simulink model "TLLTD_V1"  (R2025b)
settings: Solver=VariableStepAuto  StartTime=0.0  StopTime=10.0  RelTol=1e-3
model workspace (MAT data in the model file):
  Var = 0
  g = 9.81
values from neighbouring files (symbols this model uses):
  Track_Width = 1.00    (= 1)    [LoadTransferSimulationRevised.m]
undefined symbols (not defined in the file or in its folder): Front_Wheelbase, Rear_Wheelbase
settings Model: Creator=jakub  LastModifiedBy=jakub

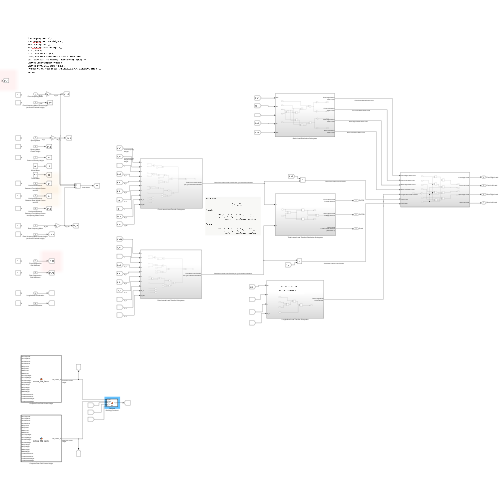
[thumbnail: Simulink's stored preview of the top-level diagram]
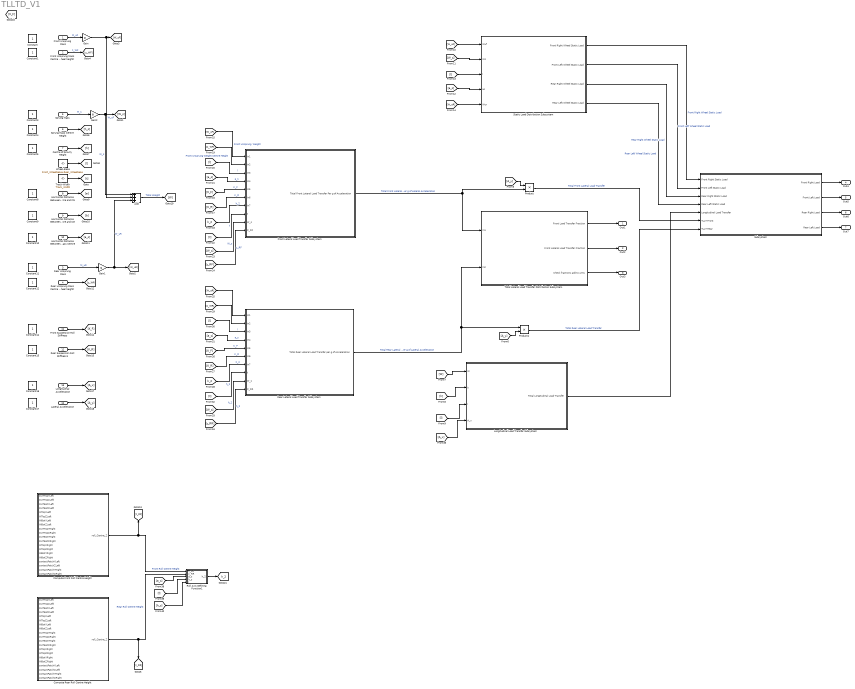
== system TLLTD_V1 ==
  Front Unsprung Mass : Inport
  Front Unsprung Mass Centre height (at centre of wheel height) : Inport  Port=2
  Rear Unsprung Mass : Inport  Port=3
  Rear Unsprung Mass Centre height (at centre of wheel height) : Inport  Port=4
  Sprung Mass : Inport  Port=5
  Sprung Mass Centre Height : Inport  Port=6
  Centre of Gravity Height : Inport  Port=7
  Horizontal Distance Between Front Wheel Centre and CG : Inport  Port=8
  Horizontal Distance Between Rear Wheel Centre and CG : Inport  Port=9
  Horizontal Distance Between Front Wheel Centre and Sprung Mass Centre : Inport  Port=10
  Front Suspension Roll Stiffness : Inport  Port=11
  Rear Suspension Roll Stiffness1 : Inport  Port=12
  Longitudinal Acceleration : Inport  Port=13
  Lateral Acceleration : Inport  Port=14
  Add : Sum  Inputs=+++
  Compute Front Roll Centre Height : MATLAB Function  TreatAsAtomicUnit=on
  Compute Rear Roll Centre Height : MATLAB Function  TreatAsAtomicUnit=on
  Constant{,1,3..5,8..12,14..17} (14 alike) : Constant
  Front Lateral Load Transfer Subsystem : Subsystem
  Gain : Gain  Gain=g
  Gain1 : Gain  Gain=g
  Gain2 : Gain  Gain=g
  Longitudinal Load Transfer Subsystem : Subsystem
  Product : Product
  Product1 : Product
  Rear Lateral Load Transfer Subsystem : Subsystem
  Roll Axis Defining Function1 : MATLAB Function  TreatAsAtomicUnit=on
  Static Load Distribution Subsystem : Subsystem
  Subsystem : Subsystem
  Total Lateral Load Transfer Distribution Subsystem : Subsystem
  Track-Width : Constant  Value=Track_Width
  Wheel-Base : Constant  Value=Front_Wheelbase+Rear_Wheelbase
  Out1 : Outport  SignalName=TLLTDF
  Out2 : Outport  Port=2  SignalName=TLLTDR
  Out3 : Outport  Port=3  SignalName=Check
  Out4 : Outport  Port=4  SignalName=Front Right Load
  Out5 : Outport  Port=5  SignalName=Front Left Load
  Out6 : Outport  Port=6  SignalName=Rear Right Load
  Out7 : Outport  Port=7  SignalName=Rear Left Load
  tag scope: h_2=global
  wires:
  Gain/1 -> Add/2, [W_uF]  "W_uF"
  Rear Unsprung Mass/1 -> Gain1/1  "M_uR"
  Gain1/1 -> Add/3, [W_uR]  "W_uR"
  Sprung Mass/1 -> Gain2/1  "M_s"
  Gain2/1 -> Add/1, [W_s]  "W_s"
  Track-Width/1 -> [t]
  Front Unsprung Mass/1 -> Gain/1  "M_uF"
  Front Unsprung Mass Centre height (at centre of wheel height)/1 -> [z_WF]  "z_WF"
  Sprung Mass Centre Height/1 -> [h_s]
  Centre of Gravity Height/1 -> [h]
  Wheel-Base/1 -> [l]
  Horizontal Distance Between Front Wheel Centre and CG/1 -> [a]
  Horizontal Distance Between Rear Wheel Centre and CG/1 -> [b]
  Horizontal Distance Between Front Wheel Centre and Sprung Mass Centre/1 -> [a_s]
  Rear Unsprung Mass Centre height (at centre of wheel height)/1 -> [z_WR]
  Front Suspension Roll Stiffness/1 -> [K_F]
  Rear Suspension Roll Stiffness1/1 -> [K_R]
  Total Lateral Load Transfer Distribution Subsystem/1(Front Load Transfer Fraction) -> Out1/1
  Total Lateral Load Transfer Distribution Subsystem/2(Front Lateral Load Transfer Fraction) -> Out2/1
  Front Lateral Load Transfer Subsystem/1(Total Front Lateral Load Transfer Per g of Acceleration) -> Total Lateral Load Transfer Distribution Subsystem/1(In1), Product/2  "Total Front Lateral Load Transfer Per g of Lateral Acceleration"
  Rear Lateral Load Transfer Subsystem/1(Total Rear Lateral Load Transfer per g of Acceleration) -> Total Lateral Load Transfer Distribution Subsystem/2(In2), Product1/1  "Total Rear Lateral Load Transfer per g of Lateral Acceleration"
  Total Lateral Load Transfer Distribution Subsystem/3(Check fractions add to unity) -> Out3/1
  Static Load Distribution Subsystem/1(Front Right Wheel Static Load) -> Subsystem/1(Front Right Static Load)  "Front Right Wheel Static Load"
  Static Load Distribution Subsystem/2(Front Left Wheel Static Load) -> Subsystem/2(Front Left Static Load)  "Front Left Wheel Static Load"
  Static Load Distribution Subsystem/3(Rear Right Wheel Static Load) -> Subsystem/3(Rear Right Static Load)  "Rear Right Wheel Static Load"
  Static Load Distribution Subsystem/4(Rear Left Wheel Static Load) -> Subsystem/4(Rear Left Static Load)  "Rear Left Wheel Static Load"
  Longitudinal Acceleration/1 -> [A_x]
  Lateral Acceleration/1 -> [A_y]
  Add/1 -> [W]  "Total Weight"
  [A_y] -> Product/1
  Product/1 -> Subsystem/6(TLLT Front)  "Total Front Lateral Load Transfer"
  [A_y] -> Product1/2
  Product1/1 -> Subsystem/7(TLLT Rear)  "Total Rear Lateral Load Transfer"
  Longitudinal Load Transfer Subsystem/1(Total Longitudinal Load Transfer) -> Subsystem/5(Longitudinal Load Transfer)
  Subsystem/1(Front Right Load) -> Out4/1
  Subsystem/2(Front Left Load) -> Out5/1
  Subsystem/3(Rear Right Load) -> Out6/1
  Subsystem/4(Rear Left Load) -> Out7/1
  [W] -> Longitudinal Load Transfer Subsystem/1(W)
  [h] -> Longitudinal Load Transfer Subsystem/2(h)
  [l] -> Longitudinal Load Transfer Subsystem/3(l)
  [W_uF] -> Static Load Distribution Subsystem/1(Wuf)
  [W_s] -> Static Load Distribution Subsystem/2(Ws)
  [l] -> Static Load Distribution Subsystem/3(l)
  [a_s] -> Static Load Distribution Subsystem/4(as)
  [W_uR] -> Static Load Distribution Subsystem/5(Wur)
  [t] -> Front Lateral Load Transfer Subsystem/8(t)  "t"
  [W_s] -> Front Lateral Load Transfer Subsystem/9(W_s)  "W_s"
  [z_RF] -> Front Lateral Load Transfer Subsystem/10(Z_RF)  "z_RF"
  [h_2] -> Front Lateral Load Transfer Subsystem/7(In7)  "h_2"
  [K_R] -> Front Lateral Load Transfer Subsystem/6(In6)  "K_R"
  [K_F] -> Front Lateral Load Transfer Subsystem/5(In5)  "K_F"
  [a_s] -> Front Lateral Load Transfer Subsystem/4(In4)  "a_s"
  [l] -> Front Lateral Load Transfer Subsystem/3(In3)  "l"
  [z_WF] -> Front Lateral Load Transfer Subsystem/2(In2)  "Front Unsprung Weight Centre Height"
  [W_uF] -> Front Lateral Load Transfer Subsystem/1(In1)  "Front Unsprung  Weight"
  [W_s] -> Rear Lateral Load Transfer Subsystem/9(W_s)  "h_2"
  [t] -> Rear Lateral Load Transfer Subsystem/8(t)  "h_2"
  [K_F] -> Rear Lateral Load Transfer Subsystem/5(In5)  "K_F"
  [h_2] -> Rear Lateral Load Transfer Subsystem/7(In7)  "h_2"
  [K_R] -> Rear Lateral Load Transfer Subsystem/6(In6)  "K_R"
  [W_uR] -> Rear Lateral Load Transfer Subsystem/1(In1)
  [a_s] -> Rear Lateral Load Transfer Subsystem/4(In4)  "a_s"
  [l] -> Rear Lateral Load Transfer Subsystem/3(In3)  "l"
  [z_RR] -> Rear Lateral Load Transfer Subsystem/10(Z_RR)  "h_2"
  [z_WR] -> Rear Lateral Load Transfer Subsystem/2(In2)
  [A_x] -> Longitudinal Load Transfer Subsystem/4(A_x)
  Compute Rear Roll Centre Height/1(roll_Centre_Z) -> [z_RR], Roll Axis Defining Function1/2(z_RR)  "Rear Roll Centre Height"
  Roll Axis Defining Function1/1(h_2) -> [h_2]
  [a_s] -> Roll Axis Defining Function1/3(a_s)
  [h_s] -> Roll Axis Defining Function1/5(l)
  [l] -> Roll Axis Defining Function1/4(h_s)
  Compute Front Roll Centre Height/1(roll_Centre_Z) -> [z_RF], Roll Axis Defining Function1/1(z_RF)  "Front Roll Centre Height"

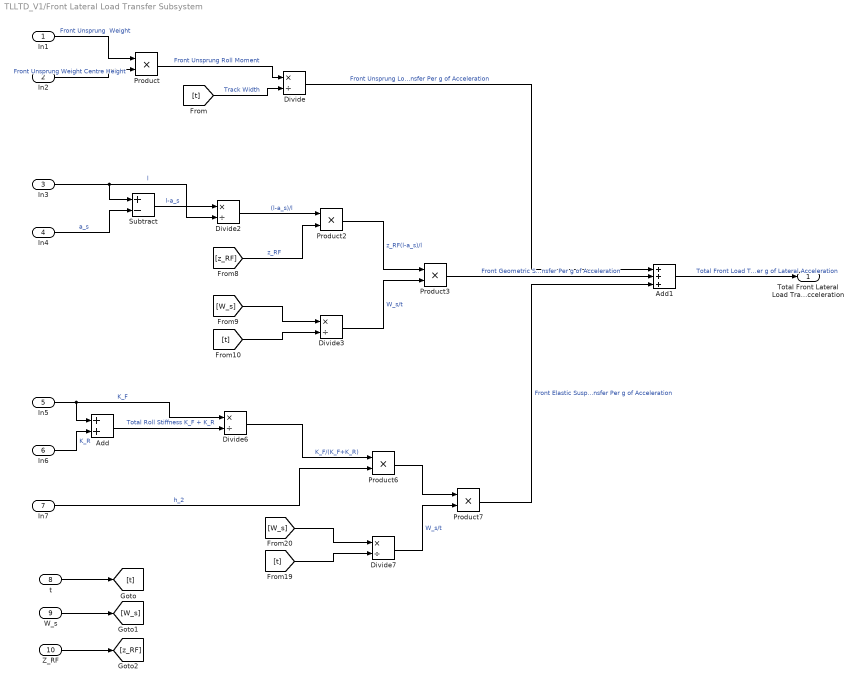
== system TLLTD_V1/Front Lateral Load Transfer Subsystem ==
  In1 : Inport
  In2 : Inport  Port=2
  In3 : Inport  Port=3
  In4 : Inport  Port=4
  In5 : Inport  Port=5
  In6 : Inport  Port=6
  In7 : Inport  Port=7
  t : Inport  Port=8
  W_s : Inport  Port=9
  Z_RF : Inport  Port=10
  Add : Sum
  Add1 : Sum  Inputs=+++
  Divide{,2..3,6..7} (5 alike) : Product  Inputs=*/
  Product{,2..3,6..7} (5 alike) : Product
  Subtract : Sum  Inputs=+-
  Total Front Lateral Load Transfer Per g of Acceleration : Outport
  wires:
  In1/1 -> Product/1  "Front Unsprung  Weight"
  Product7/1 -> Add1/3  "Front Elastic Suspended Load Transfer Per g of Acceleration"
  Divide3/1 -> Product3/2  "W_s/t"
  In2/1 -> Product/2  "Front Unsprung Weight Centre Height"
  [W_s] -> Divide3/1
  In7/1 -> Product6/2  "h_2"
  Product/1 -> Divide/1  "Front Unsprung Roll Moment"
  In3/1 -> Divide2/2, Subtract/1  "l"
  Divide/1 -> Add1/1  "Front Unsprung Load Transfer Per g of Acceleration"
  [W_s] -> Divide7/1
  In5/1 -> Divide6/1, Add/1  "K_F"
  [t] -> Divide3/2
  In4/1 -> Subtract/2  "a_s"
  [z_RF] -> Product2/2  "z_RF"
  Add/1 -> Divide6/2  "Total Roll Stiffness K_F + K_R"
  Divide2/1 -> Product2/1  "(l-a_s)/l"
  Add1/1 -> Total Front Lateral Load Transfer Per g of Acceleration/1  "Total Front Load Transfer per g of Lateral Acceleration"
  Product2/1 -> Product3/1  "z_RF(l-a_s)/l"
  Subtract/1 -> Divide2/1  "l-a_s"
  Product6/1 -> Product7/1
  [t] -> Divide7/2
  [t] -> Divide/2  "Track Width"
  Divide7/1 -> Product7/2  "W_s/t"
  Divide6/1 -> Product6/1  "K_F/(K_F+K_R)"
  In6/1 -> Add/2  "K_R"
  Product3/1 -> Add1/2  "Front Geometric Suspended Load Transfer Per g of Acceleration"
  t/1 -> [t]
  W_s/1 -> [W_s]
  Z_RF/1 -> [z_RF]

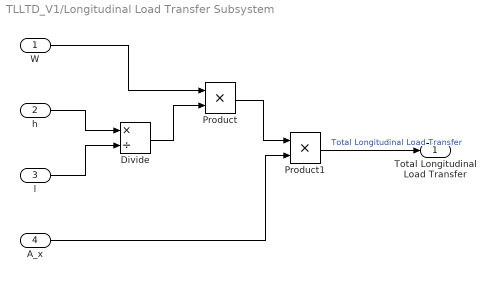
== system TLLTD_V1/Longitudinal Load Transfer Subsystem ==
  W : Inport
  h : Inport  Port=2
  l : Inport  Port=3
  A_x : Inport  Port=4
  Divide : Product  Inputs=*/
  Product : Product
  Product1 : Product
  Total Longitudinal Load Transfer : Outport
  wires:
  Product/1 -> Product1/1
  Product1/1 -> Total Longitudinal Load Transfer/1  "Total Longitudinal Load Transfer"
  Divide/1 -> Product/2
  A_x/1 -> Product1/2
  W/1 -> Product/1
  h/1 -> Divide/1
  l/1 -> Divide/2

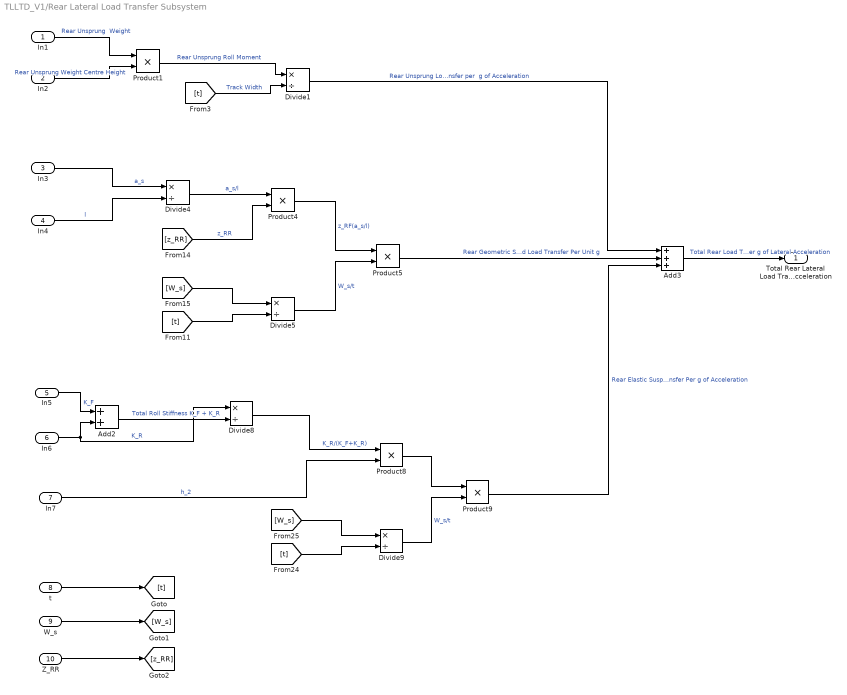
== system TLLTD_V1/Rear Lateral Load Transfer Subsystem ==
  In1 : Inport
  In2 : Inport  Port=2
  In3 : Inport  Port=3
  In4 : Inport  Port=4
  In5 : Inport  Port=5
  In6 : Inport  Port=6
  In7 : Inport  Port=7
  t : Inport  Port=8
  W_s : Inport  Port=9
  Z_RR : Inport  Port=10
  Add2 : Sum
  Add3 : Sum  Inputs=+++
  Divide{1,4..5,8..9} (5 alike) : Product  Inputs=*/
  Product{1,4..5,8..9} (5 alike) : Product
  Total Rear Lateral Load Transfer per g of Acceleration : Outport
  wires:
  Divide4/1 -> Product4/1  "a_s/l"
  Add2/1 -> Divide8/2  "Total Roll Stiffness K_F + K_R"
  [t] -> Divide9/2
  Divide8/1 -> Product8/1  "K_R/(K_F+K_R)"
  [W_s] -> Divide9/1
  Product8/1 -> Product9/1
  Add3/1 -> Total Rear Lateral Load Transfer per g of Acceleration/1  "Total Rear Load Transfer Per g of Lateral Acceleration"
  In5/1 -> Add2/1  "K_F"
  In6/1 -> Divide8/1, Add2/2  "K_R"
  Product9/1 -> Add3/3  "Rear Elastic Suspended Load Transfer Per g of Acceleration"
  In7/1 -> Product8/2  "h_2"
  Divide1/1 -> Add3/1  "Rear Unsprung Load Transfer per  g of Acceleration"
  In3/1 -> Divide4/1  "a_s"
  [t] -> Divide1/2  "Track Width"
  Product1/1 -> Divide1/1  "Rear Unsprung Roll Moment"
  In2/1 -> Product1/2  "Rear Unsprung Weight Centre Height"
  In1/1 -> Product1/1  "Rear Unsprung  Weight"
  Divide9/1 -> Product9/2  "W_s/t"
  [t] -> Divide5/2
  Product5/1 -> Add3/2  "Rear Geometric Suspended Load Transfer Per Unit g"
  [z_RR] -> Product4/2  "z_RR"
  Product4/1 -> Product5/1  "z_RF(a_s/l)"
  In4/1 -> Divide4/2  "l"
  Divide5/1 -> Product5/2  "W_s/t"
  [W_s] -> Divide5/1
  t/1 -> [t]
  W_s/1 -> [W_s]
  Z_RR/1 -> [z_RR]

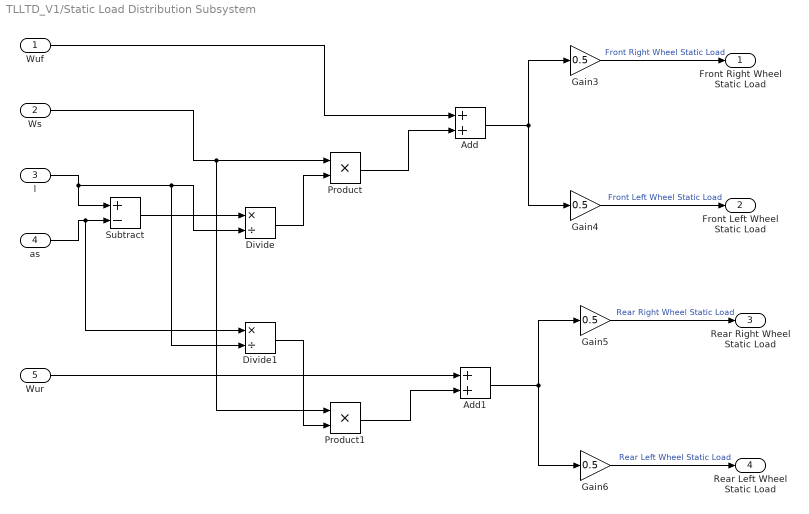
== system TLLTD_V1/Static Load Distribution Subsystem ==
  Wuf : Inport
  Ws : Inport  Port=2
  l : Inport  Port=3
  as : Inport  Port=4
  Wur : Inport  Port=5
  Add : Sum
  Add1 : Sum
  Divide : Product  Inputs=*/
  Divide1 : Product  Inputs=*/
  Gain{3..6} (4 alike) : Gain  Gain=0.5
  Product : Product
  Product1 : Product
  Subtract : Sum  Inputs=+-
  Front Right Wheel Static Load : Outport
  Front Left Wheel Static Load : Outport  Port=2
  Rear Right Wheel Static Load : Outport  Port=3
  Rear Left Wheel Static Load : Outport  Port=4
  wires:
  Gain6/1 -> Rear Left Wheel Static Load/1  "Rear Left Wheel Static Load"
  l/1 -> Divide1/2, Divide/2, Subtract/1
  Add1/1 -> Gain6/1, Gain5/1
  Product/1 -> Add/2
  Gain5/1 -> Rear Right Wheel Static Load/1  "Rear Right Wheel Static Load"
  Ws/1 -> Product1/1, Product/1
  as/1 -> Divide1/1, Subtract/2
  Add/1 -> Gain3/1, Gain4/1
  Product1/1 -> Add1/2
  Divide1/1 -> Product1/2
  Divide/1 -> Product/2
  Gain3/1 -> Front Right Wheel Static Load/1  "Front Right Wheel Static Load"
  Subtract/1 -> Divide/1
  Wuf/1 -> Add/1
  Gain4/1 -> Front Left Wheel Static Load/1  "Front Left Wheel Static Load"
  Wur/1 -> Add1/1

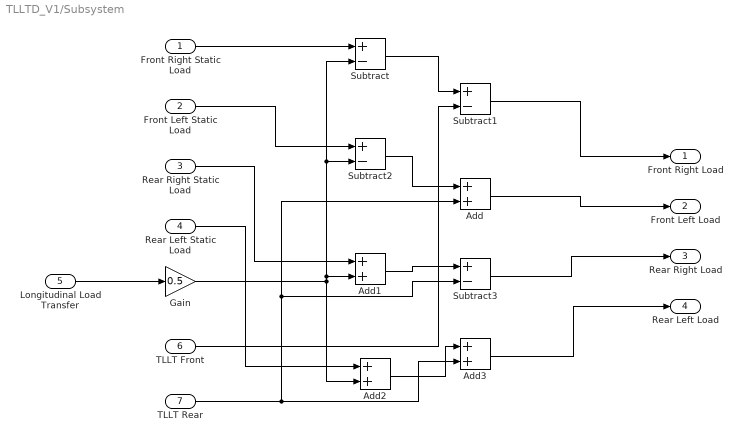
== system TLLTD_V1/Subsystem ==
  Front Right Static Load : Inport
  Front Left Static Load : Inport  Port=2
  Rear Right Static Load : Inport  Port=3
  Rear Left Static Load : Inport  Port=4
  Longitudinal Load Transfer : Inport  Port=5
  TLLT Front : Inport  Port=6
  TLLT Rear : Inport  Port=7
  Add{,1..3} (4 alike) : Sum
  Gain : Gain  Gain=0.5
  Subtract{,1..3} (4 alike) : Sum  Inputs=+-
  Front Right Load : Outport
  Front Left Load : Outport  Port=2
  Rear Right Load : Outport  Port=3
  Rear Left Load : Outport  Port=4
  wires:
  Front Right Static Load/1 -> Subtract/1
  Longitudinal Load Transfer/1 -> Gain/1
  TLLT Front/1 -> Subtract1/2
  Subtract/1 -> Subtract1/1
  Subtract1/1 -> Front Right Load/1
  Front Left Static Load/1 -> Subtract2/1
  Subtract2/1 -> Add/1
  TLLT Rear/1 -> Add3/2, Subtract3/2, Add/2
  Add/1 -> Front Left Load/1
  Rear Right Static Load/1 -> Add1/1
  Add1/1 -> Subtract3/1
  Subtract3/1 -> Rear Right Load/1
  Rear Left Static Load/1 -> Add2/1
  Add2/1 -> Add3/1
  Add3/1 -> Rear Left Load/1
  Gain/1 -> Add2/2, Subtract2/2, Subtract/2, Add1/2

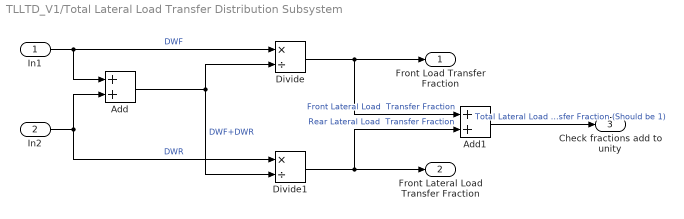
== system TLLTD_V1/Total Lateral Load Transfer Distribution Subsystem ==
  In1 : Inport
  In2 : Inport  Port=2
  Add : Sum
  Add1 : Sum
  Divide : Product  Inputs=*/
  Divide1 : Product  Inputs=*/
  Front Load Transfer Fraction : Outport
  Front Lateral Load Transfer Fraction : Outport  Port=2
  Check fractions add to unity : Outport  Port=3
  wires:
  Add1/1 -> Check fractions add to unity/1  "Total Lateral Load Transfer Fraction (Should be 1)"
  Divide1/1 -> Front Lateral Load Transfer Fraction/1, Add1/2  "Rear Lateral Load  Transfer Fraction"
  Add/1 -> Divide1/2, Divide/2  "DWF+DWR"
  Divide/1 -> Front Load Transfer Fraction/1, Add1/1  "Front Lateral Load  Transfer Fraction"
  In1/1 -> Add/1, Divide/1  "DWF"
  In2/1 -> Divide1/1, Add/2  "DWR"

== matlab function TLLTD_V1/Compute Front Roll Centre Height ==
  data: OUTTopYLeft input; roll_Centre_Z output; OUTTopZLeft input; OUTBotYLeft input; OUTBotZLeft input; INTopYLeft input; INTopZLeft input; INBotYLeft input; INBotZLeft input; OUTTopYRight input; OUTTopZRight input; OUTBotYRight input; OUTBotZRight input; INTopYRight input; INTopZRight input; INBotYRight input; INBotZRight input; contactPatchYLeft input; contactPatchZLeft input; contactPatchYRight input; contactPatchZRight input
function roll_Centre_Z = compute_Roll_Centre(OUTTopYLeft,OUTTopZLeft,OUTBotYLeft,OUTBotZLeft, ...
    INTopYLeft,INTopZLeft,INBotYLeft,INBotZLeft,OUTTopYRight,OUTTopZRight,OUTBotYRight,OUTBotZRight, ...
    INTopYRight,INTopZRight,INBotYRight,INBotZRight,contactPatchYLeft,contactPatchZLeft,contactPatchYRight, ...
    contactPatchZRight)

%Input coordinates should be relative to an origin at the FRONT LEFT TYRE
%CONTACT PATCH

%If coordinates relative to vehicle centre of gravity, coordinate
%transforms must first be done


%%%%%%%%%%%%%%%%%%%%%%%%%% LEFT INSTANT CENTRE %%%%%%%%%%%%%%%%%%%%%%%%%%%%

OUTTopLeft = [OUTTopYLeft OUTTopZLeft]
OUTBotLeft = [OUTBotYLeft OUTBotZLeft]

INTopLeft = [INTopYLeft INTopZLeft]
INBotLeft = [INBotYLeft INBotZLeft]

gradient_Top_Left = (INTopLeft(2) - OUTTopLeft(2))/(INTopLeft(1)-OUTTopLeft(1))
gradient_Bot_Left = (INBotLeft(2) - OUTBotLeft(2))/(INBotLeft(1)-OUTBotLeft(1))

inst_Centre_Y_Left = (gradient_Top_Left*OUTTopLeft(1)-gradient_Bot_Left*OUTBotLeft(1)+OUTBotLeft(2)- ...
                 OUTTopLeft(2))/(gradient_Top_Left-gradient_Bot_Left)

inst_Centre_Z_Left = gradient_Top_Left*(inst_Centre_Y_Left-OUTTopLeft(1))+OUTTopLeft(2)

%%%%%%%%%%%%%%%%%%%%%%%%%%%%%%%%%%%%%%%%%%%%%%%%%%%%%%%%%%%%%%%%%%%%%%%%%%%

%%%%%%%%%%%%%%%%%%%%%%%%%% RIGHT INSTANT CENTRE %%%%%%%%%%%%%%%%%%%%%%%%%%%

OUTTopRight = [OUTTopYRight OUTTopZRight]
OUTBotRight = [OUTBotYRight OUTBotZRight]

INTopRight = [INTopYRight INTopZRight]
INBotRight = [INBotYRight INBotZRight]

gradient_Top_Right = (INTopRight(2) - OUTTopRight(2))/(INTopRight1)-OUTTopRight(1))
gradient_Bot_Right = (INBotRight(2) - OUTBotRight(2))/(INBotRight(1)-OUTBotRight(1))

inst_Centre_Y_Right = (gradient_Top_Right*OUTTopRight(1)-gradient_Bot_Right*OUTBotRight(1)+OUTBotRight(2)- ...
                 OUTTopRight(2))/(gradient_Top_Right-gradient_Bot_Right)

inst_Centre_Z_Right = gradient_Top_Right*(inst_Centre_Y_Right-OUTTopRight(1))+OUTTopRight(2)

%%%%%%%%%%%%%%%%%%%%%%%%%%%%%%%%%%%%%%%%%%%%%%%%%%%%%%%%%%%%%%%%%%%%%%%%%%%

%%%%%%%%%%%%%%%%%%%%%%%%%% ROLL CENTRE CALCULATION %%%%%%%%%%%%%%%%%%%%%%%%

inst_Centre_Right = [inst_Centre_Y_Right inst_Centre_Z_Right]
inst_Centre_Left = [inst_Centre_Y_Left inst_Centre_Z_Left]

contact_Patch_Left = [contactPatchYLeft contactPatchZLeft]
contact_Patch_Right = [contactPatchYRight contactPatchZRight]



slope_CP_to_IC_Left = (inst_Centre_Left(2) - contact_Patch_Left(2))/(inst_Centre_Left(1)-contact_Patch_Left(1))
slope_CP_to_IC_Right = (inst_Centre_Right(2) - contact_Patch_Right(2))/(inst_Centre_Right(1)-contact_Patch_Right(1))

roll_Centre_Y = (slope_CP_to_IC_Right*inst_Centre_Right(1)-slope_CP_to_IC_Left*inst_Centre_Left(1)+inst_Centre_Left(2)- ...
                 inst_Centre_Right(2))/(slope_CP_to_IC_Right-slope_CP_to_IC_Left)

roll_Centre_Z = slope_CP_to_IC_Right*(roll_Centre_Y-inst_Centre_Right(1)) + inst_Centre_Right(2)

%%%%%%%%%%%%%%%%%%%%%%%%%%%%%%%%%%%%%%%%%%%%%%%%%%%%%%%%%%%%%%%%%%%%%%%%%%%

end

== matlab function TLLTD_V1/Compute Rear Roll Centre Height ==
  data: OUTTopYLeft input; roll_Centre_Z output; OUTTopZLeft input; OUTBotYLeft input; OUTBotZLeft input; INTopYLeft input; INTopZLeft input; INBotYLeft input; INBotZLeft input; OUTTopYRight input; OUTTopZRight input; OUTBotYRight input; OUTBotZRight input; INTopYRight input; INTopZRight input; INBotYRight input; INBotZRight input; contactPatchYLeft input; contactPatchZLeft input; contactPatchYRight input; contactPatchZRight input
function roll_Centre_Z = compute_Roll_Centre(OUTTopYLeft,OUTTopZLeft,OUTBotYLeft,OUTBotZLeft, ...
    INTopYLeft,INTopZLeft,INBotYLeft,INBotZLeft,OUTTopYRight,OUTTopZRight,OUTBotYRight,OUTBotZRight, ...
    INTopYRight,INTopZRight,INBotYRight,INBotZRight,contactPatchYLeft,contactPatchZLeft,contactPatchYRight, ...
    contactPatchZRight)

%Input coordinates should be relative to an origin at the FRONT LEFT TYRE
%CONTACT PATCH

%If coordinates relative to vehicle centre of gravity, coordinate
%transforms must first be done


%%%%%%%%%%%%%%%%%%%%%%%%%% LEFT INSTANT CENTRE %%%%%%%%%%%%%%%%%%%%%%%%%%%%

OUTTopLeft = [OUTTopYLeft OUTTopZLeft]
OUTBotLeft = [OUTBotYLeft OUTBotZLeft]

INTopLeft = [INTopYLeft INTopZLeft]
INBotLeft = [INBotYLeft INBotZLeft]

gradient_Top_Left = (INTopLeft(2) - OUTTopLeft(2))/(INTopLeft(1)-OUTTopLeft(1))
gradient_Bot_Left = (INBotLeft(2) - OUTBotLeft(2))/(INBotLeft(1)-OUTBotLeft(1))

inst_Centre_Y_Left = (gradient_Top_Left*OUTTopLeft(1)-gradient_Bot_Left*OUTBotLeft(1)+OUTBotLeft(2)- ...
                 OUTTopLeft(2))/(gradient_Top_Left-gradient_Bot_Left)

inst_Centre_Z_Left = gradient_Top_Left*(inst_Centre_Y_Left-OUTTopLeft(1))+OUTTopLeft(2)

%%%%%%%%%%%%%%%%%%%%%%%%%%%%%%%%%%%%%%%%%%%%%%%%%%%%%%%%%%%%%%%%%%%%%%%%%%%

%%%%%%%%%%%%%%%%%%%%%%%%%% RIGHT INSTANT CENTRE %%%%%%%%%%%%%%%%%%%%%%%%%%%

OUTTopRight = [OUTTopYRight OUTTopZRight]
OUTBotRight = [OUTBotYRight OUTBotZRight]

INTopRight = [INTopYRight INTopZRight]
INBotRight = [INBotYRight INBotZRight]

gradient_Top_Right = (INTopRight(2) - OUTTopRight(2))/(INTopRight1)-OUTTopRight(1))
gradient_Bot_Right = (INBotRight(2) - OUTBotRight(2))/(INBotRight(1)-OUTBotRight(1))

inst_Centre_Y_Right = (gradient_Top_Right*OUTTopRight(1)-gradient_Bot_Right*OUTBotRight(1)+OUTBotRight(2)- ...
                 OUTTopRight(2))/(gradient_Top_Right-gradient_Bot_Right)

inst_Centre_Z_Right = gradient_Top_Right*(inst_Centre_Y_Right-OUTTopRight(1))+OUTTopRight(2)

%%%%%%%%%%%%%%%%%%%%%%%%%%%%%%%%%%%%%%%%%%%%%%%%%%%%%%%%%%%%%%%%%%%%%%%%%%%

%%%%%%%%%%%%%%%%%%%%%%%%%% ROLL CENTRE CALCULATION %%%%%%%%%%%%%%%%%%%%%%%%

inst_Centre_Right = [inst_Centre_Y_Right inst_Centre_Z_Right]
inst_Centre_Left = [inst_Centre_Y_Left inst_Centre_Z_Left]

contact_Patch_Left = [contactPatchYLeft contactPatchZLeft]
contact_Patch_Right = [contactPatchYRight contactPatchZRight]



slope_CP_to_IC_Left = (inst_Centre_Left(2) - contact_Patch_Left(2))/(inst_Centre_Left(1)-contact_Patch_Left(1))
slope_CP_to_IC_Right = (inst_Centre_Right(2) - contact_Patch_Right(2))/(inst_Centre_Right(1)-contact_Patch_Right(1))

roll_Centre_Y = (slope_CP_to_IC_Right*inst_Centre_Right(1)-slope_CP_to_IC_Left*inst_Centre_Left(1)+inst_Centre_Left(2)- ...
                 inst_Centre_Right(2))/(slope_CP_to_IC_Right-slope_CP_to_IC_Left)

roll_Centre_Z = slope_CP_to_IC_Right*(roll_Centre_Y-inst_Centre_Right(1)) + inst_Centre_Right(2)

%%%%%%%%%%%%%%%%%%%%%%%%%%%%%%%%%%%%%%%%%%%%%%%%%%%%%%%%%%%%%%%%%%%%%%%%%%%

end

== matlab function TLLTD_V1/Roll Axis Defining Function1 ==
  data: z_RF input; h_2 output; z_RR input; a_s input; h_s input; l input
function h_2 = fcn(z_RF,z_RR,a_s,h_s,l)

% z_RF = Front roll centre height
% z_RR = Rear roll centre height

frontRoll = [0 z_RF]
rearRoll = [l z_RR]
sprungCentre = [a_s h_s]

NRA = rearRoll - frontRoll
NRA_Perp = -[z_RR-z_RF l]*(1/(z_RR-z_RF)^2+l^2)

FrontR_to_SprungC = sprungCentre - frontRoll
h_2 = dot(FrontR_to_SprungC,NRA_Perp)

end
